simulink subsystem "PowerSystemRefAeronomie"  (R2024b)
settings: Solver=VariableStepAuto  StartTime=0.0  StopTime=10.0  RelTol=1e-3
undefined symbols (not defined in the file or in its folder): ess, mot, powerplant, propel, pxf_diagram_options, SimIn, tc
libraries: simulink x2, slpidlib x1, matrix_library x1
(part 2 of 3)

== system PowerSystemRefAeronomie/propel/plant/parameter_selection ==
  inport-main_info_bus-1 : Inport
  Bus Selector6 : BusSelector  OutputSignals=Vehicle.EOM.AirRelativeData.Mach,Env.Atmosphere.SpeedOfSound,propel.propel_plant_speed_simu
  Constant8 : Constant  Value=mot.propel.plant.init.propD
  Gain : Gain  Gain=1/(2*pi)
  Product : Product  Inputs=*//
  Product1 : Product
  select_main_info_bus : BusSelector  OutputSignals=Env.Atmosphere.Density,tc.tc_plant_inertia_out_simu,Vehicle.EOM.InertialData.Vel_bIi,tc.tc_plant_trq_out_simu,mot.ctrl.dmd.mot_ctrl_trs_trq_simu
  outport-env_plant_density_simu-1 : Outport
  outport-tc_plant_inertia_out_simu-2 : Outport  Port=2
  outport-eqnmotion_plant_linvel_simu-3 : Outport  Port=3
  tc_plant_trq_out_simu : Outport  Port=4
  AdvanceRatio : Outport  Port=5
  wires:
  Bus Selector6/2 -> Product1/2  "<SpeedOfSound>"
  Bus Selector6/1 -> Product1/1  "<Mach>"
  Bus Selector6/3 -> Gain/1  "<propel_plant_speed_simu>"
  select_main_info_bus/4 -> tc_plant_trq_out_simu/1  "<tc_plant_trq_out_simu>"
  select_main_info_bus/1 -> outport-env_plant_density_simu-1/1  "<Density>"
  select_main_info_bus/2 -> outport-tc_plant_inertia_out_simu-2/1  "<tc_plant_inertia_out_simu>"
  select_main_info_bus/3 -> outport-eqnmotion_plant_linvel_simu-3/1  "<Vel_bIi>"
  Constant8/1 -> Product/2
  Product/1 -> AdvanceRatio/1
  inport-main_info_bus-1/1 -> select_main_info_bus/1, Bus Selector6/1
  Gain/1 -> Product/3
  Product1/1 -> Product/1

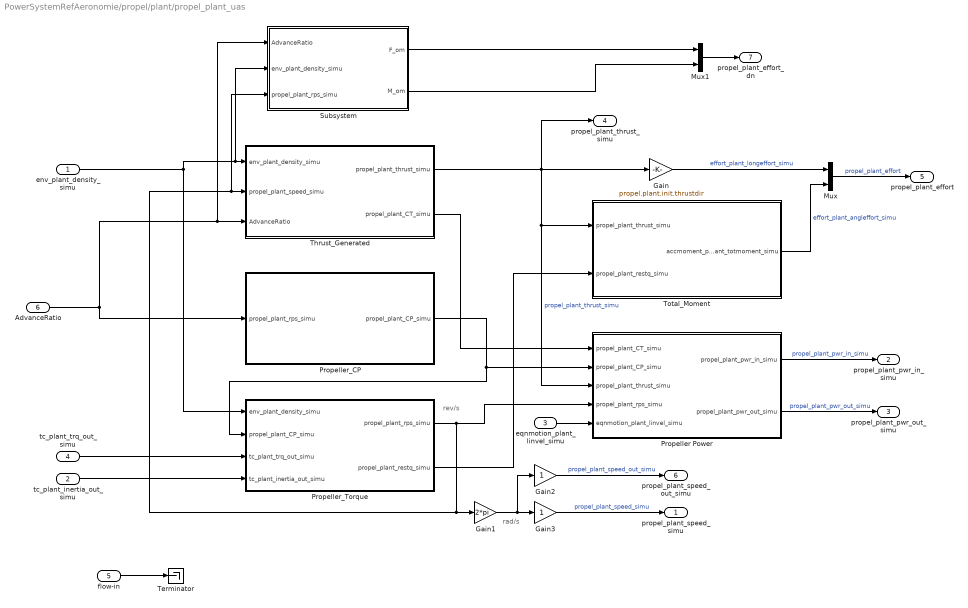
== system PowerSystemRefAeronomie/propel/plant/propel_plant_uas ==
  note: rad/s
  note: rev/s
  env_plant_density_simu : Inport
  tc_plant_inertia_out_simu : Inport  Port=2
  eqnmotion_plant_linvel_simu : Inport  Port=3
  tc_plant_trq_out_simu : Inport  Port=4
  flow-in : Inport  Port=5
  AdvanceRatio : Inport  Port=6
  Gain : Gain  Gain=propel.plant.init.thrustdir
  Gain1 : Gain  Gain=2*pi
  Gain2 : Gain
  Gain3 : Gain
  Mux : Mux  Inputs=2
  Mux1 : Mux  Inputs=2
  Propeller Power : Subsystem
  Propeller_CP : Subsystem
  Propeller_Torque : Subsystem
  Subsystem : Subsystem
  Terminator : Terminator
  Thrust_Generated : Subsystem
  Total_Moment : Subsystem
  propel_plant_speed_simu : Outport  VectorParamsAs1DForOutWhenUnconnected=off
  propel_plant_pwr_in_simu : Outport  Port=2  VectorParamsAs1DForOutWhenUnconnected=off
  propel_plant_pwr_out_simu : Outport  Port=3  VectorParamsAs1DForOutWhenUnconnected=off
  propel_plant_thrust_simu : Outport  Port=4  VectorParamsAs1DForOutWhenUnconnected=off
  propel_plant_effort : Outport  Port=5  VectorParamsAs1DForOutWhenUnconnected=off
  propel_plant_speed_out_simu : Outport  Port=6  VectorParamsAs1DForOutWhenUnconnected=off
  propel_plant_effort_dn : Outport  Port=7
  wires:
  Mux1/1 -> propel_plant_effort_dn/1
  Subsystem/2(M_om) -> Mux1/2
  Subsystem/1(F_om) -> Mux1/1
  Gain1/1 -> Gain3/1, Gain2/1
  AdvanceRatio/1 -> Propeller_CP/1(propel_plant_rps_simu), Subsystem/1(AdvanceRatio), Thrust_Generated/3(AdvanceRatio)
  flow-in/1 -> Terminator/1
  Gain3/1 -> propel_plant_speed_simu/1  "propel_plant_speed_simu"
  Gain2/1 -> propel_plant_speed_out_simu/1  "propel_plant_speed_out_simu"
  Propeller Power/1(propel_plant_pwr_in_simu) -> propel_plant_pwr_in_simu/1  "propel_plant_pwr_in_simu"
  Propeller Power/2(propel_plant_pwr_out_simu) -> propel_plant_pwr_out_simu/1  "propel_plant_pwr_out_simu"
  eqnmotion_plant_linvel_simu/1 -> Propeller Power/5(eqnmotion_plant_linvel_simu)
  Mux/1 -> propel_plant_effort/1  "propel_plant_effort"
  Gain/1 -> Mux/1  "effort_plant_longeffort_simu"
  Propeller_Torque/2(propel_plant_restq_simu) -> Total_Moment/2(propel_plant_restq_simu)
  Total_Moment/1(accmoment_plant_totmoment_simu) -> Mux/2  "effort_plant_angleffort_simu"
  tc_plant_inertia_out_simu/1 -> Propeller_Torque/4(tc_plant_inertia_out_simu)
  tc_plant_trq_out_simu/1 -> Propeller_Torque/3(tc_plant_trq_out_simu)
  env_plant_density_simu/1 -> Thrust_Generated/1(env_plant_density_simu), Subsystem/2(env_plant_density_simu), Propeller_Torque/1(env_plant_density_simu)
  Thrust_Generated/2(propel_plant_CT_simu) -> Propeller Power/1(propel_plant_CT_simu)
  Propeller_CP/1(propel_plant_CP_simu) -> Propeller Power/2(propel_plant_CP_simu), Propeller_Torque/2(propel_plant_CP_simu)
  Propeller_Torque/1(propel_plant_rps_simu) -> Gain1/1, Thrust_Generated/2(propel_plant_speed_simu), Subsystem/3(propel_plant_rps_simu), Propeller Power/4(propel_plant_rps_simu)
  Thrust_Generated/1(propel_plant_thrust_simu) -> Propeller Power/3(propel_plant_thrust_simu), Total_Moment/1(propel_plant_thrust_simu), Gain/1, propel_plant_thrust_simu/1  "propel_plant_thrust_simu"

== system PowerSystemRefAeronomie/tc/plant/parameter_out ==
  inport-tc_plant_trq_in_simu : Inport
  inport-tc_plant_trq_out_simu : Inport  Port=2
  inport-tc_plant_spd_in_simu : Inport  Port=3
  inport-tc_plant_spd_out_simu : Inport  Port=4
  inport-tc_plant_inertia_in_simu : Inport  Port=5
  inport-tc_plant_inertia_out_simu : Inport  Port=6
  Toworkspace-tc_plant_inertia_in_simu : ToWorkspace  VariableName=tc_plant_inertia_in_simu  SampleTime=pxf_diagram_options.workspace_sample_time
      settings: Decimation=pxf_diagram_options.decimation
  Toworkspace-tc_plant_inertia_out_simu : ToWorkspace  VariableName=tc_plant_inertia_out_simu  SampleTime=pxf_diagram_options.workspace_sample_time
      settings: Decimation=pxf_diagram_options.decimation
  Toworkspace-tc_plant_spd_in_simu : ToWorkspace  VariableName=tc_plant_spd_in_simu  SampleTime=pxf_diagram_options.workspace_sample_time
      settings: Decimation=pxf_diagram_options.decimation
  Toworkspace-tc_plant_spd_out_simu : ToWorkspace  VariableName=tc_plant_spd_out_simu  SampleTime=pxf_diagram_options.workspace_sample_time
      settings: Decimation=pxf_diagram_options.decimation
  Toworkspace-tc_plant_trq_in_simu : ToWorkspace  VariableName=tc_plant_trq_in_simu  SampleTime=pxf_diagram_options.workspace_sample_time
      settings: Decimation=pxf_diagram_options.decimation
  Toworkspace-tc_plant_trq_out_simu : ToWorkspace  VariableName=tc_plant_trq_out_simu  SampleTime=pxf_diagram_options.workspace_sample_time
      settings: Decimation=pxf_diagram_options.decimation
  create_system_info_bus : BusCreator  Inputs=3
  outport-system_info_bus : Outport
  wires:
  create_system_info_bus/1 -> outport-system_info_bus/1
  inport-tc_plant_trq_in_simu/1 -> Toworkspace-tc_plant_trq_in_simu/1
  inport-tc_plant_trq_out_simu/1 -> Toworkspace-tc_plant_trq_out_simu/1, create_system_info_bus/3
  inport-tc_plant_spd_in_simu/1 -> create_system_info_bus/1, Toworkspace-tc_plant_spd_in_simu/1  "tc_plant_spd_in_simu"
  inport-tc_plant_spd_out_simu/1 -> Toworkspace-tc_plant_spd_out_simu/1
  inport-tc_plant_inertia_in_simu/1 -> Toworkspace-tc_plant_inertia_in_simu/1
  inport-tc_plant_inertia_out_simu/1 -> Toworkspace-tc_plant_inertia_out_simu/1, create_system_info_bus/2  "tc_plant_inertia_out_simu"

== system PowerSystemRefAeronomie/tc/plant/parameter_selection ==

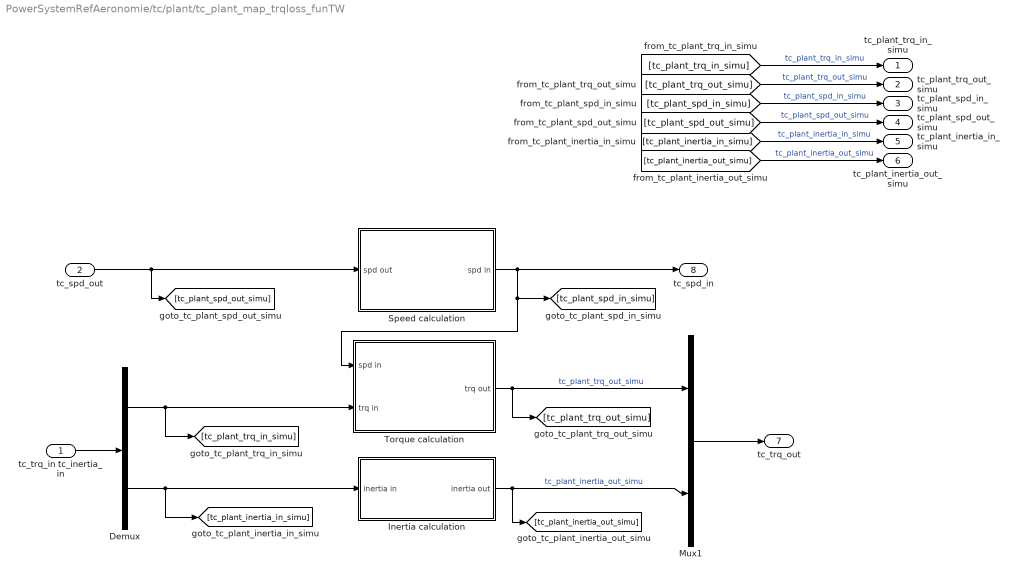
== system PowerSystemRefAeronomie/tc/plant/tc_plant_map_trqloss_funTW ==
  tc_trq_in tc_inertia_in : Inport
  tc_spd_out : Inport  Port=2
  Demux : Demux  Outputs=2
  Inertia calculation : Subsystem
  Mux1 : Mux  Inputs=2
  Speed calculation : Subsystem
  Torque calculation : Subsystem
  tc_plant_trq_in_simu : Outport
  tc_plant_trq_out_simu : Outport  Port=2
  tc_plant_spd_in_simu : Outport  Port=3
  tc_plant_spd_out_simu : Outport  Port=4
  tc_plant_inertia_in_simu : Outport  Port=5
  tc_plant_inertia_out_simu : Outport  Port=6
  tc_trq_out : Outport  Port=7
  tc_spd_in : Outport  Port=8
  wires:
  tc_trq_in tc_inertia_in/1 -> Demux/1
  Mux1/1 -> tc_trq_out/1
  [tc_plant_trq_in_simu] -> tc_plant_trq_in_simu/1  "tc_plant_trq_in_simu"
  [tc_plant_trq_out_simu] -> tc_plant_trq_out_simu/1  "tc_plant_trq_out_simu"
  [tc_plant_spd_in_simu] -> tc_plant_spd_in_simu/1  "tc_plant_spd_in_simu"
  [tc_plant_spd_out_simu] -> tc_plant_spd_out_simu/1  "tc_plant_spd_out_simu"
  [tc_plant_inertia_in_simu] -> tc_plant_inertia_in_simu/1  "tc_plant_inertia_in_simu"
  [tc_plant_inertia_out_simu] -> tc_plant_inertia_out_simu/1  "tc_plant_inertia_out_simu"
  Torque calculation/1(trq out) -> [tc_plant_trq_out_simu], Mux1/1  "tc_plant_trq_out_simu"
  Inertia calculation/1(inertia out) -> [tc_plant_inertia_out_simu], Mux1/2  "tc_plant_inertia_out_simu"
  Demux/2 -> [tc_plant_inertia_in_simu], Inertia calculation/1(inertia in)
  Demux/1 -> Torque calculation/2(trq in), [tc_plant_trq_in_simu]
  tc_spd_out/1 -> [tc_plant_spd_out_simu], Speed calculation/1(spd out)
  Speed calculation/1(spd in) -> Torque calculation/1(spd in), [tc_plant_spd_in_simu], tc_spd_in/1

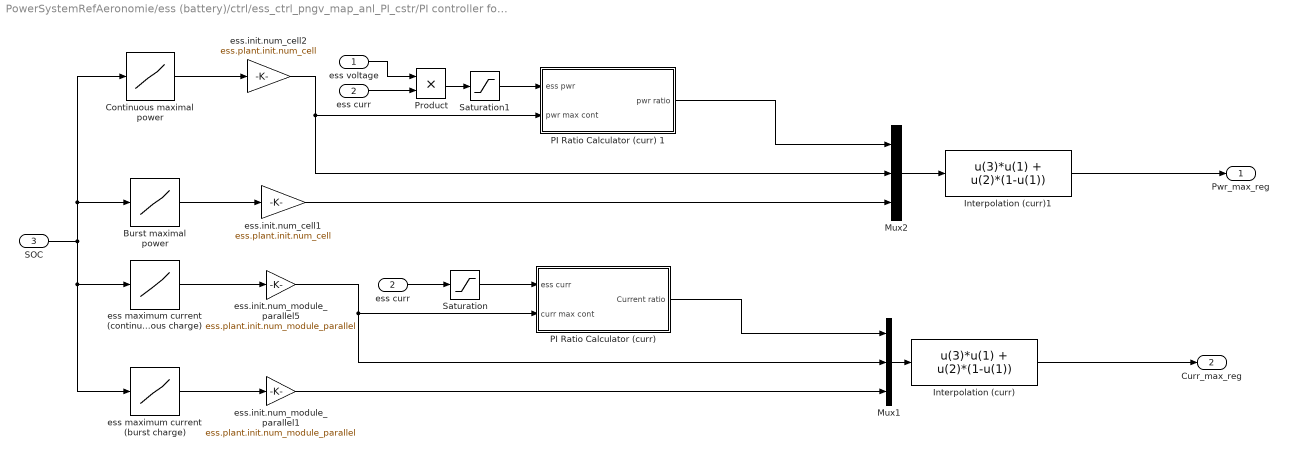
== system PowerSystemRefAeronomie/ess (battery)/ctrl/ess_ctrl_pngv_map_anl_PI_cstr/PI controller for maximal charge power and current1 ==
  ess voltage : Inport
  ess curr : Inport  Port=2
  SOC : Inport  Port=3
  Burst maximal power : Lookup  InputValues=ess.plant.init.pwr_chg_10sec.idx1_soc  Table=ess.plant.init.pwr_chg_10sec.map  SaturateOnIntegerOverflow=off
  Continuous maximal power : Lookup  InputValues=ess.plant.init.pwr_chg.idx1_soc  Table=ess.plant.init.pwr_chg.map  SaturateOnIntegerOverflow=off
  Interpolation (curr) : Fcn  Expr=u(3)*u(1) + u(2)*(1-u(1))
  Interpolation (curr)1 : Fcn  Expr=u(3)*u(1) + u(2)*(1-u(1))
  Mux1 : Mux  Inputs=3
  Mux2 : Mux  Inputs=3
  "PI Ratio Calculator (curr) " : Subsystem
  PI Ratio Calculator (curr) 1 : Subsystem
  Product : Product  RndMeth=Zero
  Saturation : Saturate  UpperLimit=0  LowerLimit=-inf
  Saturation1 : Saturate  UpperLimit=0  LowerLimit=-inf
  "ess curr " : InportShadow  Port=2
  ess maximum current (burst charge) : Lookup  InputValues=ess.plant.init.curr_chg_burst_max.idx1_soc  Table=ess.plant.init.curr_chg_burst_max.map  SaturateOnIntegerOverflow=off
  ess maximum current (continuous charge) : Lookup  InputValues=ess.plant.init.curr_chg_cont_max.idx1_soc  Table=ess.plant.init.curr_chg_cont_max.map  SaturateOnIntegerOverflow=off
  ess.init.num_cell1 : Gain  Gain=ess.plant.init.num_cell  SaturateOnIntegerOverflow=on  OutDataTypeStr=Inherit: Same as input  ParamDataTypeStr=Inherit: Same as input
  ess.init.num_cell2 : Gain  Gain=ess.plant.init.num_cell  SaturateOnIntegerOverflow=on  OutDataTypeStr=Inherit: Same as input  ParamDataTypeStr=Inherit: Same as input
  ess.init.num_module_parallel1 : Gain  Gain=ess.plant.init.num_module_parallel
  ess.init.num_module_parallel5 : Gain  Gain=ess.plant.init.num_module_parallel
  Pwr_max_reg : Outport
  Curr_max_reg : Outport  Port=2
  wires:
  ess.init.num_module_parallel1/1 -> Mux1/3
  ess.init.num_module_parallel5/1 -> "PI Ratio Calculator (curr) "/2(curr max cont), Mux1/2
  ess.init.num_cell1/1 -> Mux2/3
  ess.init.num_cell2/1 -> PI Ratio Calculator (curr) 1/2(pwr max cont), Mux2/2
  Product/1 -> Saturation1/1
  ess voltage/1 -> Product/1
  "ess curr "/1 -> Product/2
  Burst maximal power/1 -> ess.init.num_cell1/1
  PI Ratio Calculator (curr) 1/1(pwr ratio) -> Mux2/1
  Mux2/1 -> Interpolation (curr)1/1
  Interpolation (curr)1/1 -> Pwr_max_reg/1
  Continuous maximal power/1 -> ess.init.num_cell2/1
  Saturation1/1 -> PI Ratio Calculator (curr) 1/1(ess pwr)
  SOC/1 -> ess maximum current (burst charge)/1, ess maximum current (continuous charge)/1, Burst maximal power/1, Continuous maximal power/1
  Interpolation (curr)/1 -> Curr_max_reg/1
  Mux1/1 -> Interpolation (curr)/1
  ess curr/1 -> Saturation/1
  ess maximum current (continuous charge)/1 -> ess.init.num_module_parallel5/1
  ess maximum current (burst charge)/1 -> ess.init.num_module_parallel1/1
  "PI Ratio Calculator (curr) "/1(Current ratio) -> Mux1/1
  Saturation/1 -> "PI Ratio Calculator (curr) "/1(ess curr)

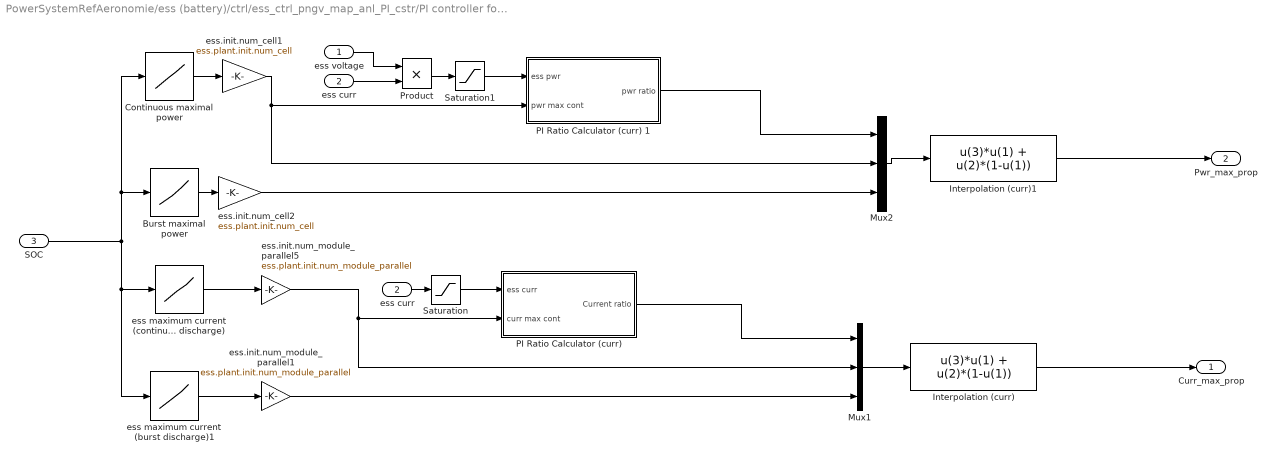
== system PowerSystemRefAeronomie/ess (battery)/ctrl/ess_ctrl_pngv_map_anl_PI_cstr/PI controller for maximal discharge power and current1 ==
  ess voltage : Inport
  ess curr : Inport  Port=2
  SOC : Inport  Port=3
  Burst maximal power : Lookup  InputValues=ess.plant.init.pwr_dis_10sec.idx1_soc  Table=ess.plant.init.pwr_dis_10sec.map  SaturateOnIntegerOverflow=off
  Continuous maximal power : Lookup  InputValues=ess.plant.init.pwr_dis.idx1_soc  Table=ess.plant.init.pwr_dis.map  SaturateOnIntegerOverflow=off
  Interpolation (curr) : Fcn  Expr=u(3)*u(1) + u(2)*(1-u(1))
  Interpolation (curr)1 : Fcn  Expr=u(3)*u(1) + u(2)*(1-u(1))
  Mux1 : Mux  Inputs=3
  Mux2 : Mux  Inputs=3
  "PI Ratio Calculator (curr) " : Subsystem
  PI Ratio Calculator (curr) 1 : Subsystem
  Product : Product  RndMeth=Zero
  Saturation : Saturate  UpperLimit=inf  LowerLimit=0
  Saturation1 : Saturate  UpperLimit=inf  LowerLimit=0
  "ess curr " : InportShadow  Port=2
  ess maximum current (burst discharge)1 : Lookup  InputValues=ess.plant.init.curr_dis_burst_max.idx1_soc  Table=ess.plant.init.curr_dis_burst_max.map  SaturateOnIntegerOverflow=off
  "ess maximum current (continuous discharge) " : Lookup  InputValues=ess.plant.init.curr_dis_cont_max.idx1_soc  Table=ess.plant.init.curr_dis_cont_max.map  SaturateOnIntegerOverflow=off
  ess.init.num_cell1 : Gain  Gain=ess.plant.init.num_cell  SaturateOnIntegerOverflow=on  OutDataTypeStr=Inherit: Same as input  ParamDataTypeStr=Inherit: Same as input
  ess.init.num_cell2 : Gain  Gain=ess.plant.init.num_cell  SaturateOnIntegerOverflow=on  OutDataTypeStr=Inherit: Same as input  ParamDataTypeStr=Inherit: Same as input
  ess.init.num_module_parallel1 : Gain  Gain=ess.plant.init.num_module_parallel
  ess.init.num_module_parallel5 : Gain  Gain=ess.plant.init.num_module_parallel
  Curr_max_prop : Outport
  Pwr_max_prop : Outport  Port=2
  wires:
  ess.init.num_module_parallel1/1 -> Mux1/3
  ess.init.num_module_parallel5/1 -> Mux1/2, "PI Ratio Calculator (curr) "/2(curr max cont)
  ess.init.num_cell2/1 -> Mux2/3
  ess.init.num_cell1/1 -> PI Ratio Calculator (curr) 1/2(pwr max cont), Mux2/2
  Product/1 -> Saturation1/1
  ess voltage/1 -> Product/1
  "ess curr "/1 -> Product/2
  Burst maximal power/1 -> ess.init.num_cell2/1
  PI Ratio Calculator (curr) 1/1(pwr ratio) -> Mux2/1
  Mux2/1 -> Interpolation (curr)1/1
  Interpolation (curr)1/1 -> Pwr_max_prop/1
  Continuous maximal power/1 -> ess.init.num_cell1/1
  Saturation1/1 -> PI Ratio Calculator (curr) 1/1(ess pwr)
  SOC/1 -> ess maximum current (burst discharge)1/1, "ess maximum current (continuous discharge) "/1, Burst maximal power/1, Continuous maximal power/1
  Saturation/1 -> "PI Ratio Calculator (curr) "/1(ess curr)
  "PI Ratio Calculator (curr) "/1(Current ratio) -> Mux1/1
  ess maximum current (burst discharge)1/1 -> ess.init.num_module_parallel1/1
  "ess maximum current (continuous discharge) "/1 -> ess.init.num_module_parallel5/1
  ess curr/1 -> Saturation/1
  Mux1/1 -> Interpolation (curr)/1
  Interpolation (curr)/1 -> Curr_max_prop/1

== system PowerSystemRefAeronomie/ess (battery)/plant/ess_plant_pngv_map_anl_PI_cstr/ess_cell ==
  ess_cell_curr : Inport
  Memory : Memory
  current polarization : Subsystem
  current polarization1 : Subsystem
  ess_soc_calculation : Subsystem
  voltage calculation : Subsystem
  ess_cell_volt_out : Outport
  ess_cell_soc : Outport  Port=2
  ess_cell_voc : Outport  Port=3
  ess_cell_rint : Outport  Port=4
  ess_cell_rpol1 : Outport  Port=5
  ess_cell_rpol2 : Outport  Port=6
  ess_cell_curr_polar2 : Outport  Port=7
  ess_cell_curr_polar1 : Outport  Port=8
  wires:
  ess_cell_curr/1 -> Memory/1
  voltage calculation/5(ess_cell_rpol2) -> ess_cell_rpol2/1
  voltage calculation/4(ess_cell_rpol1) -> ess_cell_rpol1/1
  voltage calculation/3(ess_cell_rint) -> ess_cell_rint/1
  voltage calculation/2(ess_cell_voc) -> ess_cell_voc/1
  voltage calculation/1(ess_cell_volt) -> ess_cell_volt_out/1
  current polarization1/1(ess_cell_curr_polar2) -> voltage calculation/4(ess_cell_curr_plo2), ess_cell_curr_polar2/1
  ess_soc_calculation/1(ess_soc) -> current polarization1/1(ess soc), voltage calculation/1(absolute SOC), ess_cell_soc/1, current polarization/1(ess soc)
  Memory/1 -> ess_soc_calculation/1(cell_curr), current polarization1/2(ess curr), current polarization/2(ess curr), voltage calculation/2(ess_cell_curr)
  current polarization/1(ess_cell_curr_polar1) -> voltage calculation/3(ess_cell_curr_pol1), ess_cell_curr_polar1/1

== system PowerSystemRefAeronomie/ess (battery)/plant/ess_plant_pngv_map_anl_PI_cstr/heat_generated ==
  volt_out : Inport
  ocv : Inport  Port=2
  load_current : Inport  Port=3
  Add : Sum  Inputs=-+
  Divide : Product  Inputs=*/
  Memory : Memory  InitialCondition=eps
  Product : Product  RndMeth=Zero
  square : Math  Operator=square  SignedPower=on
  heat_J : Outport
  impedance : Outport  Port=2
  wires:
  Memory/1 -> Divide/2, square/1
  Divide/1 -> impedance/1, Product/1  "R"
  Add/1 -> Divide/1
  Product/1 -> heat_J/1
  square/1 -> Product/2  "I sq"
  load_current/1 -> Memory/1
  ocv/1 -> Add/2
  volt_out/1 -> Add/1

== system PowerSystemRefAeronomie/mot/ctrl/cmd/mot_ctrl_cmd_map_Pelec_funTW_volt_in ==
  mot_plant_spd_out_simu : Inport
  mot_ctrl_trs_trq_simu : Inport  Port=2
  mot_ctrl_cstr_trq_max_pos_simu : Inport  Port=3
  mot_ctrl_cstr_trq_max_neg_simu : Inport  Port=4
  Abs : Abs
  Abs1 : Abs
  Abs2 : Abs
  Fcn : Fcn  Expr=(u>=0) - (u<0)
  Product : Product  SaturateOnIntegerOverflow=on  OutDataTypeStr=Inherit: Same as first input
  Product1 : Product  SaturateOnIntegerOverflow=on  OutDataTypeStr=Inherit: Same as first input
  Subsystem2 : Subsystem
      mask Display: disp('divider')
  Switch : Switch  InputSameDT=off
  "[-1, 1]" : Saturate  UpperLimit=1  LowerLimit=-1
  avoid zero output : Subsystem
  mot_ctrl_cmd_simu : Outport
  wires:
  avoid zero output/1(Out1) -> Product/2
  [mot_ctrl_cmd_simu] -> mot_ctrl_cmd_simu/1  "mot_ctrl_cmd_simu"
  Product1/1 -> [mot_ctrl_cmd_simu]
  mot_ctrl_cstr_trq_max_pos_simu/1 -> Abs1/1
  mot_ctrl_cstr_trq_max_neg_simu/1 -> Abs2/1
  mot_plant_spd_out_simu/1 -> avoid zero output/1(In1)
  Product/1 -> Switch/2, Fcn/1
  Switch/1 -> Subsystem2/2(In2)
  Subsystem2/1(Out1) -> "[-1, 1]"/1
  mot_ctrl_trs_trq_simu/1 -> Product/1, Abs/1
  Abs/1 -> Subsystem2/1(In1)
  Abs1/1 -> Switch/1
  Abs2/1 -> Switch/3
  "[-1, 1]"/1 -> Product1/2
  Fcn/1 -> Product1/1

== system PowerSystemRefAeronomie/mot/ctrl/cmd/parameter_out ==
  inport-mot_ctrl_cmd_simu : Inport
  Toworkspace-mot_ctrl_cmd_simu : ToWorkspace  VariableName=mot_ctrl_cmd_simu  SampleTime=pxf_diagram_options.workspace_sample_time
      settings: Decimation=pxf_diagram_options.decimation
  create_system_info_bus : BusCreator  Inputs=1
  outport-system_info_bus : Outport
  wires:
  create_system_info_bus/1 -> outport-system_info_bus/1
  inport-mot_ctrl_cmd_simu/1 -> create_system_info_bus/1, Toworkspace-mot_ctrl_cmd_simu/1  "mot_ctrl_cmd_simu"

== system PowerSystemRefAeronomie/mot/ctrl/cmd/parameter_selection ==
  inport-main_info_bus-1 : Inport
  select_main_info_bus : BusSelector  OutputSignals=mot.plant.mot_plant_spd_out_simu,mot.ctrl.dmd.mot_ctrl_trs_trq_simu,mot.ctrl.cstr.mot_ctrl_cstr_trq_max_pos_simu,mot.ctrl.cstr.mot_ctrl_cstr_trq_max_neg_simu
  outport-mot_plant_spd_out_simu-1 : Outport
  outport-mot_ctrl_trs_trq_simu-2 : Outport  Port=2
  outport-mot_ctrl_cstr_trq_max_pos_simu-3 : Outport  Port=3
  outport-mot_ctrl_cstr_trq_max_neg_simu-4 : Outport  Port=4
  wires:
  inport-main_info_bus-1/1 -> select_main_info_bus/1
  select_main_info_bus/1 -> outport-mot_plant_spd_out_simu-1/1  "<mot_plant_spd_out_simu>"
  select_main_info_bus/2 -> outport-mot_ctrl_trs_trq_simu-2/1  "<mot_ctrl_trs_trq_simu>"
  select_main_info_bus/3 -> outport-mot_ctrl_cstr_trq_max_pos_simu-3/1  "<mot_ctrl_cstr_trq_max_pos_simu>"
  select_main_info_bus/4 -> outport-mot_ctrl_cstr_trq_max_neg_simu-4/1  "<mot_ctrl_cstr_trq_max_neg_simu>"

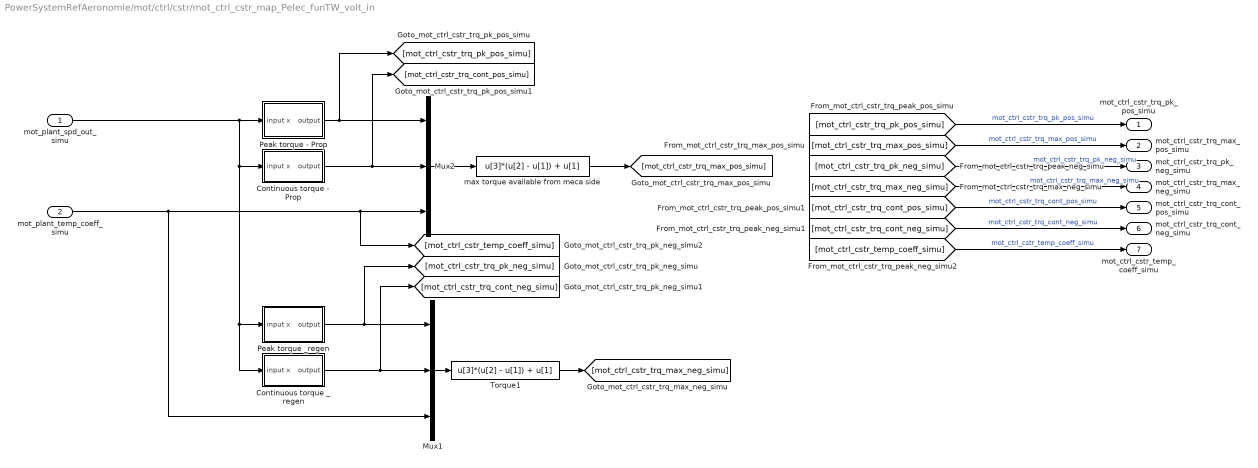
== system PowerSystemRefAeronomie/mot/ctrl/cstr/mot_ctrl_cstr_map_Pelec_funTW_volt_in ==
  mot_plant_spd_out_simu : Inport
  mot_plant_temp_coeff_simu : Inport  Port=2
  Continuous torque - Prop : Subsystem  mask{x=mot.plant.init.trq_pos_cont.idx1_spd, map=mot.plant.init.trq_pos_cont.map}
      mask Display: image(imread('map1D.jpg','jpeg'))
  Continuous torque _regen : Subsystem  mask{x=mot.plant.init.trq_neg_cont.idx1_spd, map=mot.plant.init.trq_neg_cont.map}
      mask Display: image(imread('map1D.jpg','jpeg'))
  Mux1 : Mux  Inputs=3
  Mux2 : Mux  Inputs=3
  Peak torque - Prop : Subsystem  mask{x=mot.plant.init.trq_pos_max.idx1_spd, map=mot.plant.init.trq_pos_max.map}
      mask Display: image(imread('map1D.jpg','jpeg'))
  Peak torque _regen : Subsystem  mask{x=mot.plant.init.trq_neg_max.idx1_spd, map=mot.plant.init.trq_neg_max.map}
      mask Display: image(imread('map1D.jpg','jpeg'))
  Torque1 : Fcn  Expr=u[3]*(u[2] - u[1]) + u[1]
  max torque available from meca side : Fcn  Expr=u[3]*(u[2] - u[1]) + u[1]
  mot_ctrl_cstr_trq_pk_pos_simu : Outport
  mot_ctrl_cstr_trq_max_pos_simu : Outport  Port=2
  mot_ctrl_cstr_trq_pk_neg_simu : Outport  Port=3
  mot_ctrl_cstr_trq_max_neg_simu : Outport  Port=4
  mot_ctrl_cstr_trq_cont_pos_simu : Outport  Port=5
  mot_ctrl_cstr_trq_cont_neg_simu : Outport  Port=6
  mot_ctrl_cstr_temp_coeff_simu : Outport  Port=7
  wires:
  [mot_ctrl_cstr_temp_coeff_simu] -> mot_ctrl_cstr_temp_coeff_simu/1  "mot_ctrl_cstr_temp_coeff_simu"
  [mot_ctrl_cstr_trq_cont_neg_simu] -> mot_ctrl_cstr_trq_cont_neg_simu/1  "mot_ctrl_cstr_trq_cont_neg_simu"
  [mot_ctrl_cstr_trq_cont_pos_simu] -> mot_ctrl_cstr_trq_cont_pos_simu/1  "mot_ctrl_cstr_trq_cont_pos_simu"
  [mot_ctrl_cstr_trq_pk_neg_simu] -> mot_ctrl_cstr_trq_pk_neg_simu/1  "mot_ctrl_cstr_trq_pk_neg_simu"
  [mot_ctrl_cstr_trq_max_neg_simu] -> mot_ctrl_cstr_trq_max_neg_simu/1  "mot_ctrl_cstr_trq_max_neg_simu"
  [mot_ctrl_cstr_trq_max_pos_simu] -> mot_ctrl_cstr_trq_max_pos_simu/1  "mot_ctrl_cstr_trq_max_pos_simu"
  [mot_ctrl_cstr_trq_pk_pos_simu] -> mot_ctrl_cstr_trq_pk_pos_simu/1  "mot_ctrl_cstr_trq_pk_pos_simu"
  mot_plant_spd_out_simu/1 -> Continuous torque _regen/1(input x), Peak torque _regen/1(input x), Continuous torque - Prop/1(input x), Peak torque - Prop/1(input x)
  Peak torque _regen/1(output) -> Mux1/1, [mot_ctrl_cstr_trq_pk_neg_simu]
  Peak torque - Prop/1(output) -> [mot_ctrl_cstr_trq_pk_pos_simu], Mux2/1
  mot_plant_temp_coeff_simu/1 -> [mot_ctrl_cstr_temp_coeff_simu], Mux2/3, Mux1/3
  Mux1/1 -> Torque1/1
  Continuous torque _regen/1(output) -> [mot_ctrl_cstr_trq_cont_neg_simu], Mux1/2
  Mux2/1 -> max torque available from meca side/1
  Continuous torque - Prop/1(output) -> [mot_ctrl_cstr_trq_cont_pos_simu], Mux2/2
  Torque1/1 -> [mot_ctrl_cstr_trq_max_neg_simu]
  max torque available from meca side/1 -> [mot_ctrl_cstr_trq_max_pos_simu]

== system PowerSystemRefAeronomie/mot/ctrl/cstr/parameter_out ==
  inport-mot_ctrl_cstr_trq_pk_pos_simu : Inport
  inport-mot_ctrl_cstr_trq_max_pos_simu : Inport  Port=2
  inport-mot_ctrl_cstr_trq_pk_neg_simu : Inport  Port=3
  inport-mot_ctrl_cstr_trq_max_neg_simu : Inport  Port=4
  inport-mot_ctrl_cstr_trq_cont_pos_simu : Inport  Port=5
  inport-mot_ctrl_cstr_trq_cont_neg_simu : Inport  Port=6
  inport-mot_ctrl_cstr_temp_coeff_simu : Inport  Port=7
  Ground_1 : Ground
  Toworkspace-mot_ctrl_cstr_temp_coeff_simu : ToWorkspace  VariableName=mot_ctrl_cstr_temp_coeff_simu  SampleTime=pxf_diagram_options.workspace_sample_time
      settings: Decimation=pxf_diagram_options.decimation
  Toworkspace-mot_ctrl_cstr_trq_cont_neg_simu : ToWorkspace  VariableName=mot_ctrl_cstr_trq_cont_neg_simu  SampleTime=pxf_diagram_options.workspace_sample_time
      settings: Decimation=pxf_diagram_options.decimation
  Toworkspace-mot_ctrl_cstr_trq_cont_pos_simu : ToWorkspace  VariableName=mot_ctrl_cstr_trq_cont_pos_simu  SampleTime=pxf_diagram_options.workspace_sample_time
      settings: Decimation=pxf_diagram_options.decimation
  Toworkspace-mot_ctrl_cstr_trq_max_neg_simu : ToWorkspace  VariableName=mot_ctrl_cstr_trq_max_neg_simu  SampleTime=pxf_diagram_options.workspace_sample_time
      settings: Decimation=pxf_diagram_options.decimation
  Toworkspace-mot_ctrl_cstr_trq_max_pos_simu : ToWorkspace  VariableName=mot_ctrl_cstr_trq_max_pos_simu  SampleTime=pxf_diagram_options.workspace_sample_time
      settings: Decimation=pxf_diagram_options.decimation
  Toworkspace-mot_ctrl_cstr_trq_pk_neg_simu : ToWorkspace  VariableName=mot_ctrl_cstr_trq_pk_neg_simu  SampleTime=pxf_diagram_options.workspace_sample_time
      settings: Decimation=pxf_diagram_options.decimation
  Toworkspace-mot_ctrl_cstr_trq_pk_pos_simu : ToWorkspace  VariableName=mot_ctrl_cstr_trq_pk_pos_simu  SampleTime=pxf_diagram_options.workspace_sample_time
      settings: Decimation=pxf_diagram_options.decimation
  create_system_info_bus : BusCreator  Inputs=2
  outport-system_info_bus : Outport
  outport-cstr_bus : Outport  Port=2
  wires:
  create_system_info_bus/1 -> outport-system_info_bus/1
  inport-mot_ctrl_cstr_trq_pk_pos_simu/1 -> Toworkspace-mot_ctrl_cstr_trq_pk_pos_simu/1
  inport-mot_ctrl_cstr_trq_max_pos_simu/1 -> create_system_info_bus/1, Toworkspace-mot_ctrl_cstr_trq_max_pos_simu/1  "mot_ctrl_cstr_trq_max_pos_simu"
  inport-mot_ctrl_cstr_trq_pk_neg_simu/1 -> Toworkspace-mot_ctrl_cstr_trq_pk_neg_simu/1
  inport-mot_ctrl_cstr_trq_max_neg_simu/1 -> create_system_info_bus/2, Toworkspace-mot_ctrl_cstr_trq_max_neg_simu/1  "mot_ctrl_cstr_trq_max_neg_simu"
  inport-mot_ctrl_cstr_trq_cont_pos_simu/1 -> Toworkspace-mot_ctrl_cstr_trq_cont_pos_simu/1
  inport-mot_ctrl_cstr_trq_cont_neg_simu/1 -> Toworkspace-mot_ctrl_cstr_trq_cont_neg_simu/1
  inport-mot_ctrl_cstr_temp_coeff_simu/1 -> Toworkspace-mot_ctrl_cstr_temp_coeff_simu/1
  Ground_1/1 -> outport-cstr_bus/1

== system PowerSystemRefAeronomie/mot/ctrl/cstr/parameter_selection ==
  inport-main_info_bus-1 : Inport
  select_main_info_bus : BusSelector  OutputSignals=mot.plant.mot_plant_spd_out_simu,mot.plant.mot_plant_temp_coeff_simu
  outport-mot_plant_spd_out_simu-1 : Outport
  outport-mot_plant_temp_coeff_simu-2 : Outport  Port=2
  wires:
  inport-main_info_bus-1/1 -> select_main_info_bus/1
  select_main_info_bus/1 -> outport-mot_plant_spd_out_simu-1/1  "<mot_plant_spd_out_simu>"
  select_main_info_bus/2 -> outport-mot_plant_temp_coeff_simu-2/1  "<mot_plant_temp_coeff_simu>"

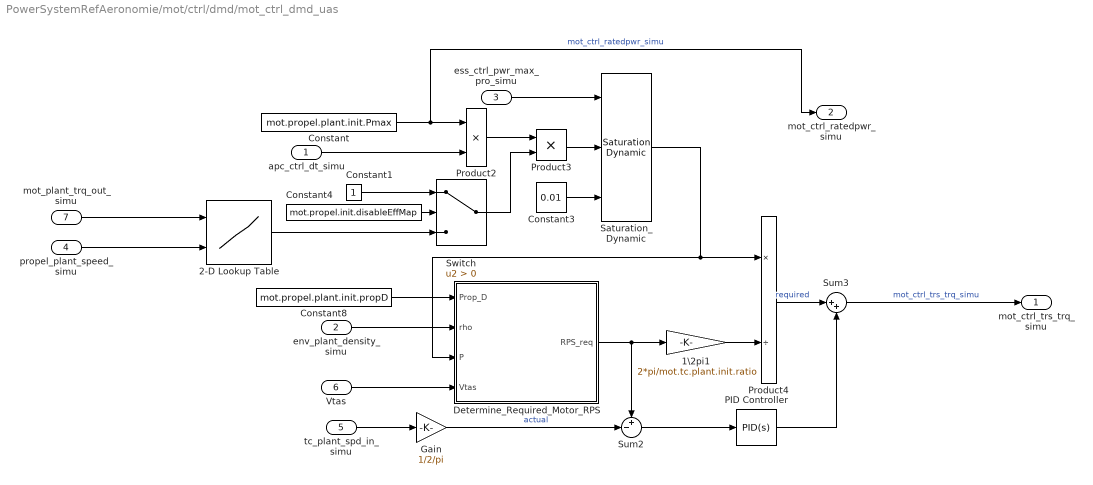
== system PowerSystemRefAeronomie/mot/ctrl/dmd/mot_ctrl_dmd_uas ==
  apc_ctrl_dt_simu : Inport
  env_plant_density_simu : Inport  Port=2
  ess_ctrl_pwr_max_pro_simu : Inport  Port=3
  propel_plant_speed_simu : Inport  Port=4
  tc_plant_spd_in_simu : Inport  Port=5
  Vtas : Inport  Port=6
  mot_plant_trq_out_simu : Inport  Port=7
  1\2pi1 : Gain  Gain=2*pi/mot.tc.plant.init.ratio
  2-D Lookup Table : Lookup_n-D  BreakpointsForDimension1=mot.plant.init.eff_trq.idx2_trq  BreakpointsForDimension2=mot.plant.init.eff_trq.idx1_spd  Table=mot.plant.init.eff_trq.map  InternalRulePriority=Speed  RndMeth=Simplest
      settings: InputPortMap=u0,u1
  Constant : Constant  Value=mot.propel.plant.init.Pmax
  Constant1 : Constant
  Constant3 : Constant  Value=0.01
  Constant4 : Constant  Value=mot.propel.init.disableEffMap
  Constant8 : Constant  Value=mot.propel.plant.init.propD
  Determine_Required_Motor_RPS : Subsystem
  Gain : Gain  Gain=1/2/pi
  PID Controller : slpidlib/PID Controller  Controller=PID  Form=Parallel  TimeDomain=Continuous-time  UseExternalTs=off  SampleTime=-1  IntegratorMethod=Forward Euler  FilterMethod=Forward Euler  ControllerParametersSource=internal  P=mot.ctrl.init.P  I=mot.ctrl.init.I  UseKiTs=off  D=mot.ctrl.init.D  UseExternalDerivativeSource=off  N=100  UseFilter=on  TunerSelectOption=Transfer Function Based (PID Tuner App)  InitialConditionSource=internal  InitialConditionForIntegrator=0  InitialConditionForFilter=0  DifferentiatorICPrevScaledInput=0  ExternalReset=none  TrackingMode=off  Kt=1  LimitOutput=off  SatLimitsSource=internal  UpperSaturationLimit=inf  LowerSaturationLimit=-inf  LinearizeAsGain=on  AntiWindupMode=none  Kb=1  LimitIntegrator=off  UpperIntegratorSaturationLimit=inf  LowerIntegratorSaturationLimit=-inf  POutMin=[]  POutMax=[]  IOutMin=[]  IOutMax=[]  DOutMin=[]  DOutMax=[]  NOutMin=[]  NOutMax=[]  SumOutMin=[]  SumOutMax=[]  SaturationOutMin=[]  SaturationOutMax=[]  PParamMin=[]  PParamMax=[]  IParamMin=[]  IParamMax=[]  DParamMin=[]  DParamMax=[]  NParamMin=[]  NParamMax=[]  KbParamMin=[]  KbParamMax=[]  KtParamMin=[]  KtParamMax=[]  KbOutMin=[]  KbOutMax=[]  KtOutMin=[]  KtOutMax=[]  IntegratorOutMin=[]  IntegratorOutMax=[]  FilterOutMin=[]  FilterOutMax=[]  SumI1OutMin=[]  SumI1OutMax=[]  SumI2OutMin=[]  SumI2OutMax=[]  SumI3OutMin=[]  SumI3OutMax=[]  SumI4OutMin=[]  SumI4OutMax=[]  SumDOutMin=[]  SumDOutMax=[]  DifferentiatorOutMin=[]  DifferentiatorOutMax=[]  FilterDiffOutCoefMin=[]  FilterDiffOutCoefMax=[]  ReciprocalOutMin=[]  ReciprocalOutMax=[]  SumDenOutMin=[]  SumDenOutMax=[]  SumNumOutMin=[]  SumNumOutMax=[]  DivideOutMin=[]  DivideOutMax=[]  UdiffTsProdOutMin=[]  UdiffTsProdOutMax=[]  NTsProdOutMin=[]  NTsProdOutMax=[]  UintegralTsProdOutMin=[]  UintegralTsProdOutMax=[]  UngainTsProdOutMin=[]  UngainTsProdOutMax=[]  ClampingZeroOutDataTypeStr=Inherit: Inherit via back propagation  ClampingZeroOutMin=[]  ClampingZeroOutMax=[]  FilterDenConstantOutDataTypeStr=Inherit: Inherit via back propagation  FilterDenConstantOutMin=[]  FilterDenConstantOutMax=[]  PCopyOutDataTypeStr=Inherit: Inherit via back propagation  PCopyOutMin=[]  PCopyOutMax=[]  NCopyOutDataTypeStr=Inherit: Inherit via back propagation  NCopyOutMin=[]  NCopyOutMax=[]  IntegratorContinuousStateAttributes=''  IntegratorStateMustResolveToSignalObject=off  IntegratorRTWStateStorageClass=Auto  FilterContinuousStateAttributes=''  FilterStateMustResolveToSignalObject=off  FilterRTWStateStorageClass=Auto  ParallelPVariant=InternalParameters  IdealPVariant=Disabled  IVariant=InternalParameters  DVariant=InternalParameters  IntegratorVariant=Continuous  SatVariant=Disabled  AWVariant=Passthrough  PCopyVariant=Disabled  TRVariant=Disabled  FdbkBlocksVariant=Forward  IdealPFdbkVariant=Disabled  SatFdbkVariant=Disabled  DerivativeFilterVariant=ContFilter  NVariant=InternalParameters  NCopyVariant=Disabled  FilterICVariant=InternalICsFilter  IntegratorICVariant=InternalICs  ExternalResetVariant=Disabled  TRSumVariant=Passthrough  SumFdbkVariant=Disabled  SumVariant=Sum_PID  TsampFilterVariant=InternalTs  TsampNgainVariant=Passthrough  TsampIntegralVariant=Disabled_SignalSpec  ExternalSaturationOutDataTypeStr=Inherit: Same as second input  DerivativeSourceVariant=ErrorSignal  PreIntVariant=InternalPreInt
  Product2 : Product  RndMeth=Zero
  Product3 : Product
  Product4 : Product  Inputs=*/  RndMeth=Zero
  Saturation_Dynamic : simulink/Discontinuities/Saturation Dynamic  OutMin=[]  OutMax=[]  OutDataTypeStr=Inherit: Same as second input  OutDataType=fixdt(1, 16)  OutScaling=2^-10  DoSatur=off
  Sum2 : Sum  Inputs=+-|
  Sum3 : Sum  Inputs=|++
  Switch : Switch  Criteria=u2 > Threshold  SaturateOnIntegerOverflow=off  InputSameDT=off
  mot_ctrl_trs_trq_simu : Outport  VectorParamsAs1DForOutWhenUnconnected=off
  mot_ctrl_ratedpwr_simu : Outport  Port=2
  wires:
  Constant4/1 -> Switch/2
  2-D Lookup Table/1 -> Switch/3
  Switch/1 -> Product3/2
  Constant1/1 -> Switch/1
  mot_plant_trq_out_simu/1 -> 2-D Lookup Table/1
  Saturation_Dynamic/1 -> Determine_Required_Motor_RPS/3(P), Product4/1
  Product3/1 -> Saturation_Dynamic/2
  Product2/1 -> Product3/1
  ess_ctrl_pwr_max_pro_simu/1 -> Saturation_Dynamic/1
  Constant3/1 -> Saturation_Dynamic/3
  Constant/1 -> mot_ctrl_ratedpwr_simu/1, Product2/1  "mot_ctrl_ratedpwr_simu"
  Vtas/1 -> Determine_Required_Motor_RPS/4(Vtas)
  env_plant_density_simu/1 -> Determine_Required_Motor_RPS/2(rho)
  Constant8/1 -> Determine_Required_Motor_RPS/1(Prop_D)
  Determine_Required_Motor_RPS/1(RPS_req) -> 1\2pi1/1, Sum2/1
  propel_plant_speed_simu/1 -> 2-D Lookup Table/2
  apc_ctrl_dt_simu/1 -> Product2/2
  Sum2/1 -> PID Controller/1
  1\2pi1/1 -> Product4/2
  Sum3/1 -> mot_ctrl_trs_trq_simu/1  "mot_ctrl_trs_trq_simu"
  PID Controller/1 -> Sum3/2
  Product4/1 -> Sum3/1  "required"
  Gain/1 -> Sum2/2  "actual"
  tc_plant_spd_in_simu/1 -> Gain/1

== system PowerSystemRefAeronomie/mot/ctrl/dmd/parameter_out ==
  inport-mot_ctrl_trs_trq_simu : Inport
  inport-mot_ctrl_ratedpwr_simu : Inport  Port=2
  Ground_1 : Ground
  Toworkspace-mot_ctrl_ratedpwr_simu : ToWorkspace  VariableName=mot_ctrl_ratedpwr_simu  SampleTime=pxf_diagram_options.workspace_sample_time
      settings: Decimation=pxf_diagram_options.decimation
  Toworkspace-mot_ctrl_trs_trq_simu : ToWorkspace  VariableName=mot_ctrl_trs_trq_simu  SampleTime=pxf_diagram_options.workspace_sample_time
      settings: Decimation=pxf_diagram_options.decimation
  create_system_info_bus : BusCreator  Inputs=1
  outport-system_info_bus : Outport
  outport-dmd_bus : Outport  Port=2
  wires:
  create_system_info_bus/1 -> outport-system_info_bus/1
  inport-mot_ctrl_trs_trq_simu/1 -> create_system_info_bus/1, Toworkspace-mot_ctrl_trs_trq_simu/1  "mot_ctrl_trs_trq_simu"
  inport-mot_ctrl_ratedpwr_simu/1 -> Toworkspace-mot_ctrl_ratedpwr_simu/1
  Ground_1/1 -> outport-dmd_bus/1

== system PowerSystemRefAeronomie/mot/ctrl/dmd/parameter_selection ==
  inport-main_info_bus-1 : Inport
  Product : Product
  Subsystem : Subsystem
  select_main_info_bus : BusSelector  OutputSignals=Cmd.EngineCmd,Env.Atmosphere.Density,ess.ctrl.ess_ctrl_pwr_max_pro_simu,propel.propel_plant_speed_simu,tc.tc_plant_spd_in_simu,Vehicle.EOM.AirRelativeData.Mach,Env.Atmosphere.SpeedOfSound,mot.plant.mot_plant_trq_out_simu
  outport-apc_ctrl_dt1_simu-1 : Outport
  outport-env_plant_density_simu-2 : Outport  Port=2
  outport-ess_ctrl_pwr_max_pro_simu-3 : Outport  Port=3
  outport-propel_plant_speed_simu-4 : Outport  Port=4
  outport-tc_plant_spd_in_simu-5 : Outport  Port=5
  Vtas : Outport  Port=6
  mot_plant_trq_out_simu : Outport  Port=7
  wires:
  select_main_info_bus/8 -> mot_plant_trq_out_simu/1  "<mot_plant_trq_out_simu>"
  Product/1 -> Vtas/1, Subsystem/3(Vtas)
  select_main_info_bus/7 -> Product/2  "<SpeedOfSound>"
  select_main_info_bus/6 -> Product/1  "<Mach>"
  Subsystem/1(EnginePwrCmd) -> outport-apc_ctrl_dt1_simu-1/1
  select_main_info_bus/1 -> Subsystem/1(<EngineCmd>)  "<EngineCmd>"
  inport-main_info_bus-1/1 -> select_main_info_bus/1
  select_main_info_bus/4 -> outport-propel_plant_speed_simu-4/1  "<propel_plant_speed_simu>"
  select_main_info_bus/5 -> outport-tc_plant_spd_in_simu-5/1  "<tc_plant_spd_in_simu>"
  select_main_info_bus/2 -> Subsystem/2(<Density>), outport-env_plant_density_simu-2/1  "<Density>"
  select_main_info_bus/3 -> outport-ess_ctrl_pwr_max_pro_simu-3/1  "<ess_ctrl_pwr_max_pro_simu>"

== system PowerSystemRefAeronomie/mot/plant/mot_plant_map_Pelec_funTW_volt_in/electric machine filter ==
  trq : Inport
  Interval Test : simulink/Logic and Bit Operations/Interval Test  IntervalClosedRight=on  uplimit=0.02  IntervalClosedLeft=on  lowlimit=-0.02  OutDataTypeStr=boolean
  Switch : Switch  Threshold=0.5  SaturateOnIntegerOverflow=off  InputSameDT=off
  electric machine time response : TransferFcn  Denominator=[mot.plant.init.time_response 1]
  filtered : Outport
  wires:
  Switch/1 -> filtered/1
  trq/1 -> electric machine time response/1, Interval Test/1, Switch/1
  Interval Test/1 -> Switch/2
  electric machine time response/1 -> Switch/3

== system PowerSystemRefAeronomie/mot/plant/mot_plant_map_Pelec_funTW_volt_in/max torque  ==
  cmd : Inport
  speed : Inport  Port=2
  torque : Inport  Port=3
  Abs : Abs
  Cont trq max - Prop : Subsystem  mask{x=mot.plant.init.trq_pos_cont.idx1_spd, map=mot.plant.init.trq_pos_cont.map}
      mask Display: image(imread('map1D.jpg','jpeg'))
  Cont trq max - Regen : Subsystem  mask{x=mot.plant.init.trq_neg_cont.idx1_spd, map=mot.plant.init.trq_neg_cont.map}
      mask Display: image(imread('map1D.jpg','jpeg'))
  Heat index : Subsystem
  Memory : Memory
  Peak trq max - Prop : Subsystem  mask{x=mot.plant.init.trq_pos_max.idx1_spd, map=mot.plant.init.trq_pos_max.map}
      mask Display: image(imread('map1D.jpg','jpeg'))
  Peak trq max - Regen : Subsystem  mask{x=mot.plant.init.trq_neg_max.idx1_spd, map=mot.plant.init.trq_neg_max.map}
      mask Display: image(imread('map1D.jpg','jpeg'))
  Product2 : Product  InputSameDT=on  SaturateOnIntegerOverflow=on  OutDataTypeStr=Inherit: Same as first input
  Product3 : Product  InputSameDT=on  SaturateOnIntegerOverflow=on  OutDataTypeStr=Inherit: Same as first input
  Product5 : Product  InputSameDT=on  SaturateOnIntegerOverflow=on  OutDataTypeStr=Inherit: Same as first input
  Sign : Signum
  Sum : Sum  InputSameDT=on  SaturateOnIntegerOverflow=on  OutDataTypeStr=Inherit: Same as first input
  Sum1 : Sum  Inputs=-+  InputSameDT=on  SaturateOnIntegerOverflow=on  OutDataTypeStr=Inherit: Same as first input
  Switch : Switch  InputSameDT=off
  Switch1 : Switch  InputSameDT=off
  cst : Constant
  max torque : Outport
  heat index : Outport  Port=2
  wires:
  Memory/1 -> Cont trq max - Prop/1(input x), Cont trq max - Regen/1(input x), Peak trq max - Regen/1(input x), Peak trq max - Prop/1(input x)
  Sign/1 -> Product5/1
  Product5/1 -> max torque/1
  Sum/1 -> Sign/1, Abs/1
  Abs/1 -> Product5/2
  torque/1 -> Heat index/2(torque)
  cmd/1 -> Switch1/2, Switch/2
  speed/1 -> Memory/1
  Cont trq max - Prop/1(output) -> Switch/1
  Cont trq max - Regen/1(output) -> Switch/3
  Peak trq max - Prop/1(output) -> Switch1/1
  Peak trq max - Regen/1(output) -> Switch1/3
  Switch/1 -> Product2/1, Heat index/1(cont torque)
  Switch1/1 -> Product3/2
  Product2/1 -> Sum/1
  Sum1/1 -> Product3/1
  Product3/1 -> Sum/2
  cst/1 -> Sum1/2
  Heat index/1(Heat index) -> Product2/2, Sum1/1, heat index/1

== system PowerSystemRefAeronomie/mot/plant/mot_plant_map_Pelec_funTW_volt_in/non-zero division ==
  note: and finally, the expression is: (u[1] \ u[2]) * 1 = u[1] \ u[2]
  note: (u[2]!=0) is true then returns 1
  note: if u[2] != 0, then output == u[1]\u[2]:
  note: (u[2]==0) is false then returns 0, thus (u[2]+(u[2]==0)) is equal to u[2]+0=u[2]
  note: and finally, the expression is: (u[1] \ 1) * 0 = 0
  note: (u[2]!=0) is false then returns 0
  note: if u[2] == 0, then output == 0:
  note: (u[2]==0) is true then returns 1, thus (u[2]+(u[2]==0)) is equal to 0+1=1
  note: original idea from Phil Sharer - ANL
      | original formula: u[1]\(u[2]+eps)*(u[2]!=0)
      | changes done by Gerald ZINI (dgey) - ANL (05\02\2001)
  In1 : Inport
  In2 : Inport  Port=2
  Fcn : Fcn  Expr=u[1]/(u[2]+(u[2]==0))*(u[2]!=0)
  Mux : Mux  Inputs=2
  Out1 : Outport
  wires:
  In2/1 -> Mux/2
  Fcn/1 -> Out1/1
  In1/1 -> Mux/1
  Mux/1 -> Fcn/1

== system PowerSystemRefAeronomie/propel/plant/propel_plant_uas/Propeller Power ==
  propel_plant_CT_simu : Inport
  propel_plant_CP_simu : Inport  Port=2
  propel_plant_thrust_simu : Inport  Port=3
  propel_plant_rps_simu : Inport  Port=4
  eqnmotion_plant_linvel_simu : Inport  Port=5
  Dot Product : DotProduct  OutDataTypeStr=Inherit: Inherit via internal rule
  Fcn : Fcn  Expr=u(2) / u(1) * u(4) * u(3) * propel.plant.init.propD
  Mux : Mux
  Product : Product
  Sqrt : Sqrt
  propel_plant_pwr_in_simu : Outport  VectorParamsAs1DForOutWhenUnconnected=off
  propel_plant_pwr_out_simu : Outport  Port=2  VectorParamsAs1DForOutWhenUnconnected=off
  wires:
  Dot Product/1 -> Sqrt/1
  eqnmotion_plant_linvel_simu/1 -> Dot Product/1, Dot Product/2
  Sqrt/1 -> Product/2  "tas"
  Product/1 -> propel_plant_pwr_out_simu/1
  Mux/1 -> Fcn/1
  propel_plant_CT_simu/1 -> Mux/1
  propel_plant_thrust_simu/1 -> Mux/3, Product/1
  propel_plant_rps_simu/1 -> Mux/4
  Fcn/1 -> propel_plant_pwr_in_simu/1  "propel_plant_pwr_in_simu"
  propel_plant_CP_simu/1 -> Mux/2

== system PowerSystemRefAeronomie/propel/plant/propel_plant_uas/Propeller_CP ==
  propel_plant_rps_simu : Inport
  CP : Polyval  Coefs=powerplant.propel.init.CPpoly
  propel_plant_CP_simu : Outport  VectorParamsAs1DForOutWhenUnconnected=off
  wires:
  propel_plant_rps_simu/1 -> CP/1
  CP/1 -> propel_plant_CP_simu/1

== system PowerSystemRefAeronomie/propel/plant/propel_plant_uas/Propeller_Torque ==
  note: I = Wprop*R^2/3g
      | General Aviation Aircraft Design pg 619
  env_plant_density_simu : Inport
  propel_plant_CP_simu : Inport  Port=2
  tc_plant_trq_out_simu : Inport  Port=3
  tc_plant_inertia_out_simu : Inport  Port=4
  " " : Gain  Gain=-1
  "2pi " : Gain  Gain=1/2/pi
  Fcn1 : Fcn  Expr=(u(1)/(2*pi)) *u(3)*(u(2)^2)*(propel.plant.init.propD^5)
  Integrator1 : Integrator  InitialCondition=propel.ctrl.init.rps
  Mux : Mux  Inputs=3
  Product : Product  Inputs=*/
  Prop Inertia : Constant  Value=propel.plant.init.Iprop
  Sum1 : Sum  Inputs=|+-
  Sum2 : Sum  Inputs=|++
  propel_plant_rps_simu : Outport  VectorParamsAs1DForOutWhenUnconnected=off
  propel_plant_restq_simu : Outport  Port=2  VectorParamsAs1DForOutWhenUnconnected=off
  wires:
  tc_plant_trq_out_simu/1 -> Sum1/1
  "2pi "/1 -> Integrator1/1
  Mux/1 -> Fcn1/1
  " "/1 -> propel_plant_restq_simu/1
  Integrator1/1 -> propel_plant_rps_simu/1, Mux/2  "propeller_plant_rps_simu"
  env_plant_density_simu/1 -> Mux/3  "env_plant_density_simu"
  propel_plant_CP_simu/1 -> Mux/1  "prop_plant_CP_simu"
  Fcn1/1 -> Sum1/2, " "/1  "propel_plant_restq_simu"
  Prop Inertia/1 -> Sum2/1
  tc_plant_inertia_out_simu/1 -> Sum2/2
  Sum2/1 -> Product/2
  Sum1/1 -> Product/1
  Product/1 -> "2pi "/1

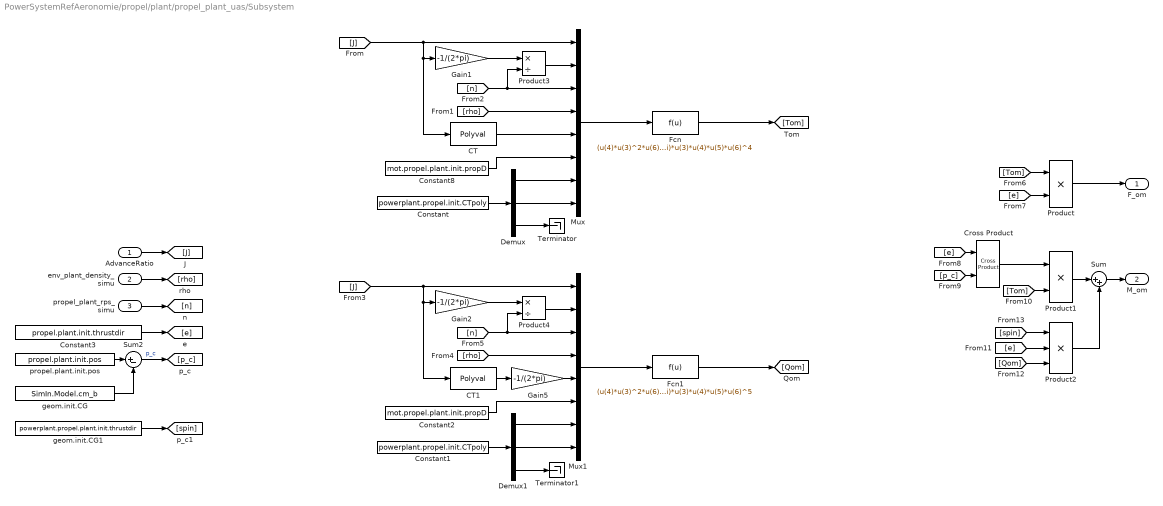
== system PowerSystemRefAeronomie/propel/plant/propel_plant_uas/Subsystem ==
  AdvanceRatio : Inport
  env_plant_density_simu : Inport  Port=2
  propel_plant_rps_simu : Inport  Port=3
  CT : Polyval  Coefs=powerplant.propel.init.CTpoly
  CT1 : Polyval  Coefs=powerplant.propel.init.CTpoly
  Constant : Constant  Value=powerplant.propel.init.CTpoly
  Constant1 : Constant  Value=powerplant.propel.init.CTpoly
  Constant2 : Constant  Value=mot.propel.plant.init.propD
  Constant3 : Constant  Value=propel.plant.init.thrustdir
  Constant8 : Constant  Value=mot.propel.plant.init.propD
  Cross Product : matrix_library/Cross Product
  Demux : Demux  Outputs=3
  Demux1 : Demux  Outputs=3
  Fcn : Fcn  Expr=(u(4)*u(3)^2*u(6)^4)*(2*u(7)*u(1)+u(8))*(u(2))+(1/pi)*u(3)*u(4)*u(5)*u(6)^4
  Fcn1 : Fcn  Expr=(u(4)*u(3)^2*u(6)^5)*(-(2*u(7)*u(1)+u(8))/pi)*(u(2))+(1/pi)*u(3)*u(4)*u(5)*u(6)^5
  Gain1 : Gain  Gain=-1/(2*pi)
  Gain2 : Gain  Gain=-1/(2*pi)
  Gain5 : Gain  Gain=-1/(2*pi)
  Mux : Mux  Inputs=8
  Mux1 : Mux  Inputs=8
  Product : Product
  Product1 : Product
  Product2 : Product  Inputs=3
  Product3 : Product  Inputs=*/
  Product4 : Product  Inputs=*/
  Sum : Sum  Inputs=|++
  Sum2 : Sum  Inputs=|+-  SaturateOnIntegerOverflow=on
  Terminator : Terminator
  Terminator1 : Terminator
  geom.init.CG : Constant  Value=SimIn.Model.cm_b
  geom.init.CG1 : Constant  Value=powerplant.propel.plant.init.thrustdir
  propel.plant.init.pos : Constant  Value=propel.plant.init.pos
  F_om : Outport
  M_om : Outport  Port=2
  wires:
  Gain5/1 -> Mux1/5
  CT1/1 -> Gain5/1
  Mux1/1 -> Fcn1/1
  Demux1/2 -> Mux1/8
  [n] -> Product4/2, Mux1/3
  Constant1/1 -> Demux1/1
  Demux1/3 -> Terminator1/1
  Gain2/1 -> Product4/1
  Constant2/1 -> Mux1/6
  [J] -> Gain2/1, CT1/1, Mux1/1
  Demux1/1 -> Mux1/7
  Product4/1 -> Mux1/2
  [rho] -> Mux1/4
  Constant8/1 -> Mux/6
  Demux/2 -> Mux/8
  Demux/1 -> Mux/7
  CT/1 -> Mux/5
  [rho] -> Mux/4
  Product3/1 -> Mux/2
  Gain1/1 -> Product3/1
  [spin] -> Product2/1
  geom.init.CG1/1 -> [spin]
  Sum/1 -> M_om/1
  Product2/1 -> Sum/2
  [Qom] -> Product2/3
  [e] -> Product2/2
  [Tom] -> Product1/2
  Cross Product/1 -> Product1/1
  Product1/1 -> Sum/1
  [p_c] -> Cross Product/2
  [e] -> Cross Product/1
  [e] -> Product/2
  [Tom] -> Product/1
  Product/1 -> F_om/1
  geom.init.CG/1 -> Sum2/2
  propel.plant.init.pos/1 -> Sum2/1
  Sum2/1 -> [p_c]  "p_c"
  Constant3/1 -> [e]
  propel_plant_rps_simu/1 -> [n]
  env_plant_density_simu/1 -> [rho]
  AdvanceRatio/1 -> [J]
  Fcn1/1 -> [Qom]
  Demux/3 -> Terminator/1
  Constant/1 -> Demux/1
  Mux/1 -> Fcn/1
  Fcn/1 -> [Tom]
  [n] -> Product3/2, Mux/3
  [J] -> Gain1/1, CT/1, Mux/1

== system PowerSystemRefAeronomie/propel/plant/propel_plant_uas/Thrust_Generated ==
  env_plant_density_simu : Inport
  propel_plant_speed_simu : Inport  Port=2
  AdvanceRatio : Inport  Port=3
  CT : Polyval  Coefs=powerplant.propel.init.CTpoly
  Mux5 : Mux  Inputs=3
  RPS2T : Fcn  Expr=u(2) * u(3) * propel.plant.init.propD^4 * u(1)^2
  propel_plant_thrust_simu : Outport  VectorParamsAs1DForOutWhenUnconnected=off
  propel_plant_CT_simu : Outport  Port=2  VectorParamsAs1DForOutWhenUnconnected=off
  wires:
  AdvanceRatio/1 -> CT/1
  CT/1 -> Mux5/2, propel_plant_CT_simu/1
  env_plant_density_simu/1 -> Mux5/3
  propel_plant_speed_simu/1 -> Mux5/1
  Mux5/1 -> RPS2T/1
  RPS2T/1 -> propel_plant_thrust_simu/1

== system PowerSystemRefAeronomie/propel/plant/propel_plant_uas/Total_Moment ==
  propel_plant_thrust_simu : Inport
  propel_plant_restq_simu : Inport  Port=2
  Gain : Gain  Gain=propel.plant.init.rotationdir
  Gain1 : Gain  Gain=propel.plant.init.thrustdir
  Gain2 : Gain  Gain=propel.plant.init.thrustdir  Multiplication=Matrix(K*u) (u vector)
  Moment_due_to_eng_position : Subsystem
  Sum2 : Sum  Inputs=|+-  SaturateOnIntegerOverflow=on
  Sum4 : Sum  SaturateOnIntegerOverflow=on
  geom.init.CG : Constant  Value=SimIn.Model.cm_b
  propel.plant.init.pos : Constant  Value=propel.plant.init.pos
  accmoment_plant_totmoment_simu : Outport  VectorParamsAs1DForOutWhenUnconnected=off
  wires:
  Gain2/1 -> Sum4/2
  propel_plant_restq_simu/1 -> Gain/1
  Gain1/1 -> Moment_due_to_eng_position/2(Vec 2)
  Gain/1 -> Gain2/1
  Sum2/1 -> Moment_due_to_eng_position/1(Vec 1)
  Sum4/1 -> accmoment_plant_totmoment_simu/1  "accmoment_plant_totmoment_simu"
  propel.plant.init.pos/1 -> Sum2/1
  geom.init.CG/1 -> Sum2/2
  propel_plant_thrust_simu/1 -> Gain1/1
  Moment_due_to_eng_position/1(X Prod) -> Sum4/1

== system PowerSystemRefAeronomie/tc/plant/tc_plant_map_trqloss_funTW/Inertia calculation ==
  inertia in : Inport
  Sum3 : Sum  Inputs=|++  InputSameDT=on  SaturateOnIntegerOverflow=on  OutDataTypeStr=Inherit: Same as first input
  tc inertia : Constant  Value=tc.plant.init.inertia
  tc.plant.init.ratio : Gain  Gain=tc.plant.init.ratio
  "tc.plant.init.ratio " : Gain  Gain=tc.plant.init.ratio
  inertia out : Outport
  wires:
  "tc.plant.init.ratio "/1 -> tc.plant.init.ratio/1
  inertia in/1 -> "tc.plant.init.ratio "/1
  tc.plant.init.ratio/1 -> Sum3/1
  tc inertia/1 -> Sum3/2
  Sum3/1 -> inertia out/1

== system PowerSystemRefAeronomie/tc/plant/tc_plant_map_trqloss_funTW/Speed calculation ==
  spd out : Inport
  tc.plant.init.ratio : Gain  Gain=tc.plant.init.ratio
  spd in : Outport
  wires:
  spd out/1 -> tc.plant.init.ratio/1
  tc.plant.init.ratio/1 -> spd in/1

== system PowerSystemRefAeronomie/tc/plant/tc_plant_map_trqloss_funTW/Torque calculation ==
  spd in : Inport
  trq in : Inport  Port=2
  Abs : Abs
  Abs1 : Abs
  Blending (state dependent) : Subsystem  mask(State dependent blending){xl=-tc.plant.init.spd_thresh, yl=-1, xc=0, yc=0, xr=tc.plant.init.spd_thresh, yr=1}
      mask prompts: xl "Left point (x):"; yl "Left point (y):"; xc "Center point (x):"; yc "Center point (y):"; xr "Right point (x):"; yr "Right point (y):"
      mask help: This block implements state dependent smoothing/blending. IMPORTANT: See help menu.
      mask Help: The output equals the product of the first input and a "hat" function defined by the three points specified in the dialog box.  The second input forms the argument to the hat function.\n\nIMPORTANT: A divide by zero error will result if first coordinates of the three points specified for the hat function are NOT distinct.
      mask Display: plot([-1 1 3 6 8], [1.5 1.5 0.5 4.0 4.0])
  Sum2 : Sum  Inputs=|+-  InputSameDT=on  SaturateOnIntegerOverflow=on  OutDataTypeStr=Inherit: Same as first input
  tc.plant.init.ratio : Gain  Gain=tc.plant.init.ratio
  trq losses : Subsystem  mask(Lookup Table (2-D)){x=tc.plant.init.trq_loss.idx1_trq, y=tc.plant.init.trq_loss.idx2_spd, t=tc.plant.init.trq_loss.map}
      mask prompts: x "Row:"; y "Column:"; t "Table:"
      mask help: Performs 2-D linear interpolation of input values using the specified input/output table. Extrapolation is performed outside the table boundaries.
      mask init:
      | [r,c]=size(t);
      | xt=reshape(x,prod(size(x)),1);
      | xi=xt(:,ones(1,c));
      | minx=min(x); maxx=max(x);
      | mint=min(min(t)); maxt=max(max(t));
      mask Display: plot(xi,t,[minx maxx],[mint mint],[minx minx],[mint maxt])
  trq out : Outport
  wires:
  tc.plant.init.ratio/1 -> trq out/1
  Sum2/1 -> tc.plant.init.ratio/1
  trq in/1 -> Sum2/1, Abs/1
  spd in/1 -> Blending (state dependent)/2(Control (state)), Abs1/1
  Blending (state dependent)/1(Output) -> Sum2/2
  trq losses/1(Out1) -> Blending (state dependent)/1(Input)
  Abs1/1 -> trq losses/2(Cols)
  Abs/1 -> trq losses/1(Rows)

== system PowerSystemRefAeronomie/ess (battery)/ctrl/ess_ctrl_pngv_map_anl_PI_cstr/PI controller for maximal charge power and current1/PI Ratio Calculator (curr)  ==
  note: %deviation
  ess curr : Inport
  curr max cont : Inport  Port=2
  Add1 : Sum  Inputs=-+
  Integrator1 : Integrator  InitialCondition=ess.plant.init.ul_curr_chg  LimitOutput=on  UpperSaturationLimit=ess.plant.init.ul_curr_chg  LowerSaturationLimit=ess.plant.init.ll_curr_chg
  Ki_curr : Gain  Gain=ess.plant.init.Ki_curr_chg  SaturateOnIntegerOverflow=on  OutDataTypeStr=Inherit: Same as input  ParamDataTypeStr=Inherit: Same as input
  Saturation1 : Saturate  UpperLimit=1  LowerLimit=0
  non-zero division1 : Subsystem
      mask Display: disp('divider')
  Current ratio : Outport
  wires:
  Add1/1 -> non-zero division1/1(In1)
  non-zero division1/1(Out1) -> Ki_curr/1
  Ki_curr/1 -> Integrator1/1
  Integrator1/1 -> Saturation1/1
  ess curr/1 -> Add1/1
  Saturation1/1 -> Current ratio/1
  curr max cont/1 -> Add1/2, non-zero division1/2(In2)
